simulink model "AircraftModel"  (R2025b)
settings: Solver=VariableStepAuto  StartTime=0.0  StopTime=200  RelTol=1e-3
InitFcn:
  | load("Aero.mat");
  | load("Prop.mat");
  | load("Motor.mat")
values from neighbouring files (symbols this model uses):
  A =     [Aero.mat]    (also in Aerodynamic.m = evalin("base", 'A'); QuaternionKinematics.m = [[0 -w(1) -w(2) -w(3)]; RotationalDynamics.m = evalin("base", "A"))
  Prop =     [Prop.mat]    (also in Propulsion.m = evalin("base", 'Prop'))
  WindAxes = [Va;a;b]    [Aerodynamic.m]
undefined symbols (not defined in the file or in its folder): Aerodynamic, Coordinates, Euler2Qbi, Euler2Rbi, EulerKinematics, Propulsion, Qbi2Euler, Qbi2Rbi, QuaternionKinematics, RotationalDynamics, WGS84
libraries: matrix_library x3, aerolibfltsims x2, simulink x1, aerolibatmos2 x1, sharedutil x1, aerosimlib x1
settings Model: Creator=User  LastModifiedBy=sutur
settings RTWCC: GPUComputeCapability=3.5

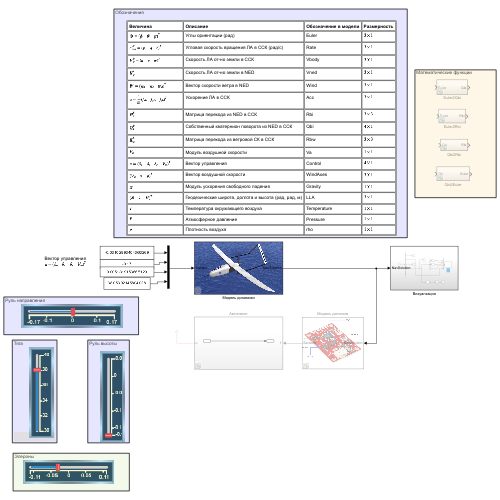
[thumbnail: Simulink's stored preview of the top-level diagram]
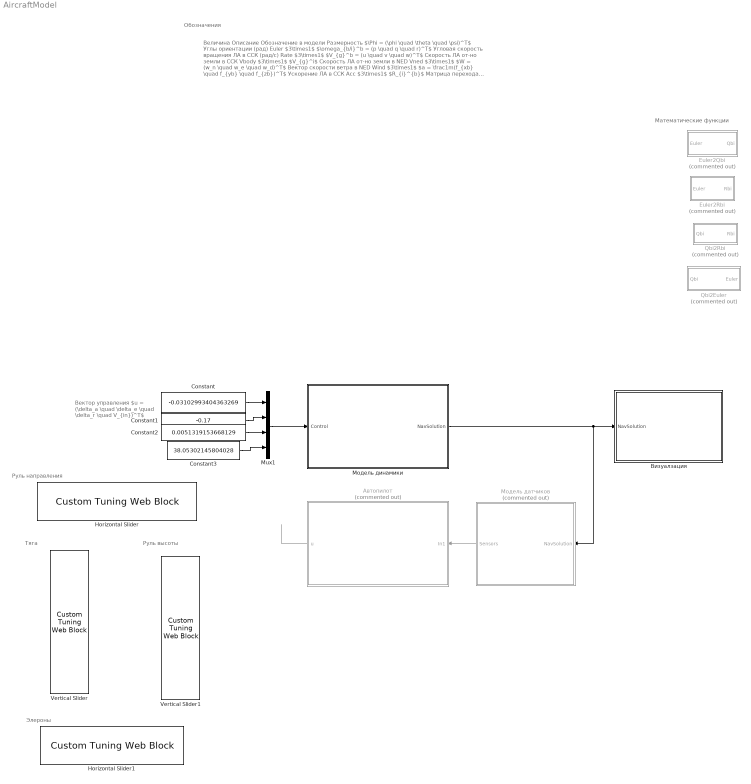
== system AircraftModel ==
  note: Руль направления
  note: Элероны
  note: Руль высоты
  note: Тяга
  note: Вектор управления
      | $u = (\delta_a \quad \delta_e \quad \delta_r \quad V_{in})^T$
  note: Математические функции
  note: Величина
      | Описание
      | Обозначение в модели
      | Размерность
      |
      | $\Phi = (\phi \quad \theta \quad \psi)^T$
      | Углы ориентации (рад)
      | Euler
      | $3\times1$
      |
      | $\omega_{b/i}^b = (p \quad q \quad r)^T$
      | Угловая скорость вращения ЛА в ССК (рад/с)
      | Rate
      | $3\times1$
      |
      | $V_{g}^b = (u \quad v \quad w)^T$
      | Скорость ЛА от-но земли в ССК
      | Vbody
      | $3\times1$
      |
      | $V_{g}^i$
      | Скорость ЛА от-но земли в NED
      | Vned
      | $3\times1$
      |
      | $W = (w_n \quad w_e \quad w_d)^T$
      | Вектор скорости ветра в NED
      | Wind
      | $3\times1$
      |
      | $a = \frac1m(f_{xb} \quad f_{yb} \quad f_{zb})^T$
      | Ускорение ЛА в ССК
      | Acc
      | $3\times1$
      |
      | $R_{i}^{b}$
      | Матрица перехода из NED в ССК
      | Rbi
      | $3\times3$
      |
      | $Q_{i}^{b}$
      | Собственный кватернион поворота из NED в ССК
      | Qbi
      | $4\times1$
      |
      | $R_w^b$
      | Матрица перехода из ветровой СК в ССК
      | Rbw
      | $3\times3$
      |
      | $V_a$
      | Модуль воздушной скорости
      | Va
      | $1\times1$
      |
      | $u = (\delta_a \quad \delta_e \quad \delta_r \quad V_{in})^T$
      | Вектор управления
      | Control
      | $4\times1$
      |
      | $(V_a \quad \alpha \quad \beta)^T$
      | Вектор воздушной скорости
      | WindAxes
      | $3\times1$
      |
      | $g$
      | Модуль ускорения свободного падения
      | Gravity
      | $1\times1$
      |
      | $(\phi \quad \lambda \quad H)^T$
      | Геодезические широта, долгота и высота (рад, рад, м)
      | LLA
      | $3\times1$
      |
      | $T$
      | Температура окружающего воздуха
      | Temperature
      | $1\times1$
      |
      | $P$
      | Атмосферное давление
      | Pressure
      | $1\times1$
      |
      | $\rho$
      | Плотность воздуха
      | rho
      | $1\times1$
  note: Обозначения
  Constant : Constant  Value=-0.03102993404363269
  Constant1 : Constant  Value=-0.17
  Constant2 : Constant  Value=0.0051319153668129
  Constant3 : Constant  Value=38.05302145804028
  Euler2Qbi : Subsystem  Commented=on
  Euler2Rbi : Subsystem  Commented=on
  Horizontal Slider : CustomTuningWebBlock  LabelPosition=Hide  ShowInitialText=on  Configuration="{\"components\":[{\"name\":\"LinearScaleComponent\",\"settings\":{\"bounds\":{\"max\":0.17,\"min\":-0.17,\"tickInterval\":\"auto\"},\"internalTickHeightScaleFactor\":0.5,\"labelColor\":[255,255,200],\"labelFont\":{\"font\":\"Arial\",\"fontSize\":12},\"labelOffset\":0.05,\"labelTransparency\":1,\"needleImage\":{\"size\":[596,842],\"src\":\"data:image\\/svg+xml;base64,PD94bWwgdmVyc2lvbj0iMS4wIiBlbmNvZGluZz0idXRmLTgiPz4NCjwhLS0gR2VuZXJhdG9yOiBBZG9iZSBJbGx1c3RyYXRvciAyNS4wLjAsIFNWRyBFeHBvcnQgUGx1Zy1JbiAuIFNWRyBWZXJzaW9uOiA2LjAwIEJ1aWxkIDApICAtLT4NCjxzdmcgdmVyc2lvbj0iMS4xIg0KCSBpZD0ic3ZnOCIgeG1sbnM6Y2M9Imh0dHA6Ly9jcmVhdGl2ZWNvbW1vbnMub3JnL25zIyIgeG1sbnM6ZGM9Imh0dHA6Ly9wdXJsLm9yZy9kYy9lbGVtZW50cy8xLjEvIiB4bWxuczppbmtzY2FwZT0iaHR0cDovL3d3dy5pbmtzY2FwZS5vcmcvbmFtZXNw ...(+2420 chars)\",\"srcOrientation\":\"Right\"},\"needleOffset\":[-0.8044596912521441,-0.0642123287671233],\"needleSize\":{\"height\":0.4337797619047619,\"width\":0.07668067226890757},\"position\":[0.2829861111111111,0.04398634453781513,0.9196428571428571,0.6088789682539683],\"referencePoint\":\"auto\",\"scaleColors\":[],\"scaleColorsSize\":0.2,\"scaleDirection\":\"LR\",\"showLabels\":1,\"showMinorTicks\":0,\"showSpanLine\":1,\"showTicks\":1,\"tickColor\":[252,252,197],\"tickTransparency\":1,\"valueBarColor\":[0,114,189],\"valueBarOffset\":-0.27,\"valueBarSize\":0.1,\"valueBarTransparency\":1}},{\"name\":\"BackgroundImageComponent\",\"settings\":{\"image\":{\"size\":[380,101],\"src\":\"data:image\\/svg+xml;base64,PHN2ZyB4bWxucz0iaHR0cDovL3d3dy53My5vcmcvMjAwMC9zdmciIHhtbG5zOnhsaW5rPSJodHRwOi8vd3d3LnczLm9yZy8xOTk5L3hsaW5rIiB2aWV3Qm94PSIwIDAgMzgwIDEwMSI+PGRlZnM+PHN0eWxlPi5jbHMtMXtmaWxsOiMwMDJiNDI7fS5jbHMtMntmaWxsOiM0MjcwODI7fS5jbHMtM3tmaWxsOnVybCgjcmFkaWFsLWdyYWRpZW50KTt9LmNscy00e2ZpbGw6I2M4YzhjODtzdHJva2U6IzAwMDt9PC9zdHlsZT48cmFkaWFsR3JhZGllbnQgaWQ9InJhZGlhbC1ncmFkaWVudCIgY3g9IjE5MCIgY3k9IjUwLjUiIHI9IjI2OS4yMSIgZ3JhZGllbnRVbml0cz0idXNlclNwYWNlT25Vc2UiPjxzdG9wIG9mZnNldD0iMC4wMSIgc3RvcC1jb2xvcj0iIzNlNGY1OCIvPjxzdG9wIG9mZnNldD0iMC4wNiIgc3RvcC1jb2xvcj0iIzQ0NTc2MSIvPjxzdG9wIG9mZnNldD0iMC4xNSIgc3RvcC1jb2xvcj0iIzU1NmE3NiIvPjxzdG9wIG9mZnNldD0iMC4yNSIgc3RvcC1jb2xvcj0iIzZkODg5NSIvPjxzdG9wIG9mZnNldD0iMC4zOCIgc3RvcC1jb2xvcj0iIzhmYjJjMyIvPjxzdG9wIG9mZnNldD0iMC41MiIgc3RvcC1jb2xvcj0iI2I2ZTRmYSIvPjxzdG9wIG9mZnNldD0iMSIgc3RvcC1jb2xvcj0iIzE1NDY1NyIvPjwvcmFkaWFsR3JhZGllbnQ+PC9kZWZzPjxnIGlkPSJmcmFtZSI+PGcgaWQ9IkxheWVyXzIiIGRhdGEtbmFtZT0iTGF5ZXIgMiI+PGcgaWQ9IkxheWVyXzEtMiIgZGF0YS1uYW1lPSJMYXllciAxLTIiPjxyZWN0IGlkPSJyZWN0MTAzNiIgY2xhc3M9ImNscy0xIiB4PSIxMSIgeT0iMTEiIHdpZHRoPSIzNTgiIGhlaWdodD0iNzkiLz48cGF0aCBpZD0icGF0aDEwMzgiIGNsYXNzPSJjbHMtMiIgZD0iTTgsOFY5M0gzNzJWOFpNMzY5LDkwSDExVjExSDM2OVoiLz48cGF0aCBpZD0icGF0aDEwNDAiIGNsYXNzPSJjbHMtMyIgZD0iTTAsMFYxMDFIMzgwVjBaTTM3Miw5M0g4VjhIMzcyWiIvPjwvZz48L2c+PC9nPjxnIGlkPSJ0cmFjayI+PHBhdGggaWQ9InJlY3QxNjExIiBjbGFzcz0iY2xzLTQiIGQ9Ik0zMy4zNywyNi41OUgzNDYuNjNjNCwwLDcuMjUsMi42LDcuMjUsNS44MWgwYzAsMy4yMS0zLjI1LDUuODItNy4yNSw1LjgySDMzLjM3Yy00LDAtNy4yNS0yLjYxLTcuMjUtNS44MmgwQzI2LjEyLDI5LjE5LDI5LjM3LDI2LjU5LDMzLjM3LDI2LjU5WiIvPjwvZz48L3N2Zz4=\",\"srcOrientation\":\"horizontal\"},\"position\":[0,0,1,1],\"scaleMode\":\"0\"}},{\"name\":\"ForegroundImageComponent\",\"settings\":{\"image\":{\"size\":[0,0],\"src\":\"default\",\"srcOrientation\":[]},\"isForeground\":1,\"position\":[0,0,1,1],\"scaleMode\":\"0\"}}],\"derived\":{\"blockParameters\":{\"ForegroundColor\":[0.9882352941176471,0.9882352941176471,0.7725490196078432],\"Limits\":{\"Max\":0.17,\"Min\":-0.17,\"Ticks\":\"auto\"},\"ScaleColors\":[],\"ScaleDirection\":\"Clockwise\",\"ScaleMax\":0.17,\"ScaleMin\":-0.17,\"TickInterval\":\"auto\",\"fixedAspectRatio\":\"on\"}},\"settings\":{\"BindingType\":\"param\",\"aspectRatio\":3.7777777777777777,\"backgroundColor\":[0,0,0,\"1\"],\"backgroundOffset\":0,\"backgroundOpacity\":1,\"fixedAspectRatio\":\"on\",\"foregroundColor\":[252,252,196],\"orientation\":\"horizontal\",\"showBackgroundColor\":false,\"value\":0,\"version\":\"R2023a\"},\"type\":\"LinearGauge\"}"
  Horizontal Slider1 : CustomTuningWebBlock  LabelPosition=Hide  ShowInitialText=on  Configuration="{\"components\":[{\"name\":\"LinearScaleComponent\",\"settings\":{\"bounds\":{\"max\":0.11,\"min\":-0.11,\"tickInterval\":\"auto\"},\"internalTickHeightScaleFactor\":0.5,\"labelColor\":[255,255,200],\"labelFont\":{\"font\":\"Arial\",\"fontSize\":12},\"labelOffset\":0.05,\"labelTransparency\":1,\"needleImage\":{\"size\":[596,842],\"src\":\"data:image\\/svg+xml;base64,PD94bWwgdmVyc2lvbj0iMS4wIiBlbmNvZGluZz0idXRmLTgiPz4NCjwhLS0gR2VuZXJhdG9yOiBBZG9iZSBJbGx1c3RyYXRvciAyNS4wLjAsIFNWRyBFeHBvcnQgUGx1Zy1JbiAuIFNWRyBWZXJzaW9uOiA2LjAwIEJ1aWxkIDApICAtLT4NCjxzdmcgdmVyc2lvbj0iMS4xIg0KCSBpZD0ic3ZnOCIgeG1sbnM6Y2M9Imh0dHA6Ly9jcmVhdGl2ZWNvbW1vbnMub3JnL25zIyIgeG1sbnM6ZGM9Imh0dHA6Ly9wdXJsLm9yZy9kYy9lbGVtZW50cy8xLjEvIiB4bWxuczppbmtzY2FwZT0iaHR0cDovL3d3dy5pbmtzY2FwZS5vcmcvbmFtZXNw ...(+2420 chars)\",\"srcOrientation\":\"Right\"},\"needleOffset\":[-0.8044596912521441,-0.0642123287671233],\"needleSize\":{\"height\":0.4337797619047619,\"width\":0.07668067226890757},\"position\":[0.2829861111111111,0.04398634453781513,0.9196428571428571,0.6088789682539683],\"referencePoint\":\"auto\",\"scaleColors\":[],\"scaleColorsSize\":0.2,\"scaleDirection\":\"LR\",\"showLabels\":1,\"showMinorTicks\":0,\"showSpanLine\":1,\"showTicks\":1,\"tickColor\":[252,252,197],\"tickTransparency\":1,\"valueBarColor\":[0,114,189],\"valueBarOffset\":-0.27,\"valueBarSize\":0.1,\"valueBarTransparency\":1}},{\"name\":\"BackgroundImageComponent\",\"settings\":{\"image\":{\"size\":[380,101],\"src\":\"data:image\\/svg+xml;base64,PHN2ZyB4bWxucz0iaHR0cDovL3d3dy53My5vcmcvMjAwMC9zdmciIHhtbG5zOnhsaW5rPSJodHRwOi8vd3d3LnczLm9yZy8xOTk5L3hsaW5rIiB2aWV3Qm94PSIwIDAgMzgwIDEwMSI+PGRlZnM+PHN0eWxlPi5jbHMtMXtmaWxsOiMwMDJiNDI7fS5jbHMtMntmaWxsOiM0MjcwODI7fS5jbHMtM3tmaWxsOnVybCgjcmFkaWFsLWdyYWRpZW50KTt9LmNscy00e2ZpbGw6I2M4YzhjODtzdHJva2U6IzAwMDt9PC9zdHlsZT48cmFkaWFsR3JhZGllbnQgaWQ9InJhZGlhbC1ncmFkaWVudCIgY3g9IjE5MCIgY3k9IjUwLjUiIHI9IjI2OS4yMSIgZ3JhZGllbnRVbml0cz0idXNlclNwYWNlT25Vc2UiPjxzdG9wIG9mZnNldD0iMC4wMSIgc3RvcC1jb2xvcj0iIzNlNGY1OCIvPjxzdG9wIG9mZnNldD0iMC4wNiIgc3RvcC1jb2xvcj0iIzQ0NTc2MSIvPjxzdG9wIG9mZnNldD0iMC4xNSIgc3RvcC1jb2xvcj0iIzU1NmE3NiIvPjxzdG9wIG9mZnNldD0iMC4yNSIgc3RvcC1jb2xvcj0iIzZkODg5NSIvPjxzdG9wIG9mZnNldD0iMC4zOCIgc3RvcC1jb2xvcj0iIzhmYjJjMyIvPjxzdG9wIG9mZnNldD0iMC41MiIgc3RvcC1jb2xvcj0iI2I2ZTRmYSIvPjxzdG9wIG9mZnNldD0iMSIgc3RvcC1jb2xvcj0iIzE1NDY1NyIvPjwvcmFkaWFsR3JhZGllbnQ+PC9kZWZzPjxnIGlkPSJmcmFtZSI+PGcgaWQ9IkxheWVyXzIiIGRhdGEtbmFtZT0iTGF5ZXIgMiI+PGcgaWQ9IkxheWVyXzEtMiIgZGF0YS1uYW1lPSJMYXllciAxLTIiPjxyZWN0IGlkPSJyZWN0MTAzNiIgY2xhc3M9ImNscy0xIiB4PSIxMSIgeT0iMTEiIHdpZHRoPSIzNTgiIGhlaWdodD0iNzkiLz48cGF0aCBpZD0icGF0aDEwMzgiIGNsYXNzPSJjbHMtMiIgZD0iTTgsOFY5M0gzNzJWOFpNMzY5LDkwSDExVjExSDM2OVoiLz48cGF0aCBpZD0icGF0aDEwNDAiIGNsYXNzPSJjbHMtMyIgZD0iTTAsMFYxMDFIMzgwVjBaTTM3Miw5M0g4VjhIMzcyWiIvPjwvZz48L2c+PC9nPjxnIGlkPSJ0cmFjayI+PHBhdGggaWQ9InJlY3QxNjExIiBjbGFzcz0iY2xzLTQiIGQ9Ik0zMy4zNywyNi41OUgzNDYuNjNjNCwwLDcuMjUsMi42LDcuMjUsNS44MWgwYzAsMy4yMS0zLjI1LDUuODItNy4yNSw1LjgySDMzLjM3Yy00LDAtNy4yNS0yLjYxLTcuMjUtNS44MmgwQzI2LjEyLDI5LjE5LDI5LjM3LDI2LjU5LDMzLjM3LDI2LjU5WiIvPjwvZz48L3N2Zz4=\",\"srcOrientation\":\"horizontal\"},\"position\":[0,0,1,1],\"scaleMode\":\"0\"}},{\"name\":\"ForegroundImageComponent\",\"settings\":{\"image\":{\"size\":[0,0],\"src\":\"default\",\"srcOrientation\":[]},\"isForeground\":1,\"position\":[0,0,1,1],\"scaleMode\":\"0\"}}],\"derived\":{\"blockParameters\":{\"ForegroundColor\":[0.9882352941176471,0.9882352941176471,0.7725490196078432],\"Limits\":{\"Max\":0.11,\"Min\":-0.11,\"Ticks\":\"auto\"},\"ScaleColors\":[],\"ScaleDirection\":\"Clockwise\",\"ScaleMax\":0.11,\"ScaleMin\":-0.11,\"TickInterval\":\"auto\",\"fixedAspectRatio\":\"on\"}},\"settings\":{\"BindingType\":\"param\",\"aspectRatio\":3.7777777777777777,\"backgroundColor\":[0,0,0,\"1\"],\"backgroundOffset\":0,\"backgroundOpacity\":1,\"fixedAspectRatio\":\"on\",\"foregroundColor\":[252,252,196],\"orientation\":\"horizontal\",\"showBackgroundColor\":false,\"value\":0,\"version\":\"R2023a\"},\"type\":\"LinearGauge\"}"
  Mux1 : Mux
  Qbi2Euler : Subsystem  Commented=on
  Qbi2Rbi : Subsystem  Commented=on
  Vertical Slider : CustomTuningWebBlock  LabelPosition=Hide  ShowInitialText=on  Configuration="{\"components\":[{\"name\":\"LinearScaleComponent\",\"settings\":{\"bounds\":{\"max\":40,\"min\":30,\"tickInterval\":\"auto\"},\"internalTickHeightScaleFactor\":0.5,\"labelColor\":[255,255,200],\"labelFont\":{\"font\":\"Arial\",\"fontSize\":12},\"labelOffset\":0.05,\"labelTransparency\":1,\"needleImage\":{\"size\":[596,842],\"src\":\"data:image\\/svg+xml;base64,PD94bWwgdmVyc2lvbj0iMS4wIiBlbmNvZGluZz0idXRmLTgiPz4NCjwhLS0gR2VuZXJhdG9yOiBBZG9iZSBJbGx1c3RyYXRvciAyNS4wLjAsIFNWRyBFeHBvcnQgUGx1Zy1JbiAuIFNWRyBWZXJzaW9uOiA2LjAwIEJ1aWxkIDApICAtLT4NCjxzdmcgdmVyc2lvbj0iMS4xIg0KCSBpZD0ic3ZnOCIgeG1sbnM6Y2M9Imh0dHA6Ly9jcmVhdGl2ZWNvbW1vbnMub3JnL25zIyIgeG1sbnM6ZGM9Imh0dHA6Ly9wdXJsLm9yZy9kYy9lbGVtZW50cy8xLjEvIiB4bWxuczppbmtzY2FwZT0iaHR0cDovL3d3dy5pbmtzY2FwZS5vcmcvbmFtZXNw ...(+2420 chars)\",\"srcOrientation\":\"horizontal\"},\"needleOffset\":[0.0642123287671233,-0.8044596912521441],\"needleSize\":{\"height\":0.07668067226890757,\"width\":0.4337797619047619},\"position\":[0.03623949579831933,0.2829861111111111,0.6088789682539683,0.9196428571428571],\"referencePoint\":\"auto\",\"scaleColors\":[],\"scaleColorsSize\":0.2,\"scaleDirection\":\"BT\",\"showLabels\":1,\"showMinorTicks\":0,\"showSpanLine\":1,\"showTicks\":1,\"tickColor\":[252,252,197],\"tickTransparency\":1,\"valueBarColor\":[0,114,189],\"valueBarOffset\":-0.27,\"valueBarSize\":0.1,\"valueBarTransparency\":1}},{\"name\":\"BackgroundImageComponent\",\"settings\":{\"image\":{\"size\":[380,101],\"src\":\"data:image\\/svg+xml;base64,PHN2ZyB4bWxucz0iaHR0cDovL3d3dy53My5vcmcvMjAwMC9zdmciIHhtbG5zOnhsaW5rPSJodHRwOi8vd3d3LnczLm9yZy8xOTk5L3hsaW5rIiB2aWV3Qm94PSIwIDAgMzgwIDEwMSI+PGRlZnM+PHN0eWxlPi5jbHMtMXtmaWxsOiMwMDJiNDI7fS5jbHMtMntmaWxsOiM0MjcwODI7fS5jbHMtM3tmaWxsOnVybCgjcmFkaWFsLWdyYWRpZW50KTt9LmNscy00e2ZpbGw6I2M4YzhjODtzdHJva2U6IzAwMDt9PC9zdHlsZT48cmFkaWFsR3JhZGllbnQgaWQ9InJhZGlhbC1ncmFkaWVudCIgY3g9IjE5MCIgY3k9IjUwLjUiIHI9IjI2OS4yMSIgZ3JhZGllbnRVbml0cz0idXNlclNwYWNlT25Vc2UiPjxzdG9wIG9mZnNldD0iMC4wMSIgc3RvcC1jb2xvcj0iIzNlNGY1OCIvPjxzdG9wIG9mZnNldD0iMC4wNiIgc3RvcC1jb2xvcj0iIzQ0NTc2MSIvPjxzdG9wIG9mZnNldD0iMC4xNSIgc3RvcC1jb2xvcj0iIzU1NmE3NiIvPjxzdG9wIG9mZnNldD0iMC4yNSIgc3RvcC1jb2xvcj0iIzZkODg5NSIvPjxzdG9wIG9mZnNldD0iMC4zOCIgc3RvcC1jb2xvcj0iIzhmYjJjMyIvPjxzdG9wIG9mZnNldD0iMC41MiIgc3RvcC1jb2xvcj0iI2I2ZTRmYSIvPjxzdG9wIG9mZnNldD0iMSIgc3RvcC1jb2xvcj0iIzE1NDY1NyIvPjwvcmFkaWFsR3JhZGllbnQ+PC9kZWZzPjxnIGlkPSJmcmFtZSI+PGcgaWQ9IkxheWVyXzIiIGRhdGEtbmFtZT0iTGF5ZXIgMiI+PGcgaWQ9IkxheWVyXzEtMiIgZGF0YS1uYW1lPSJMYXllciAxLTIiPjxyZWN0IGlkPSJyZWN0MTAzNiIgY2xhc3M9ImNscy0xIiB4PSIxMSIgeT0iMTEiIHdpZHRoPSIzNTgiIGhlaWdodD0iNzkiLz48cGF0aCBpZD0icGF0aDEwMzgiIGNsYXNzPSJjbHMtMiIgZD0iTTgsOFY5M0gzNzJWOFpNMzY5LDkwSDExVjExSDM2OVoiLz48cGF0aCBpZD0icGF0aDEwNDAiIGNsYXNzPSJjbHMtMyIgZD0iTTAsMFYxMDFIMzgwVjBaTTM3Miw5M0g4VjhIMzcyWiIvPjwvZz48L2c+PC9nPjxnIGlkPSJ0cmFjayI+PHBhdGggaWQ9InJlY3QxNjExIiBjbGFzcz0iY2xzLTQiIGQ9Ik0zMy4zNywyNi41OUgzNDYuNjNjNCwwLDcuMjUsMi42LDcuMjUsNS44MWgwYzAsMy4yMS0zLjI1LDUuODItNy4yNSw1LjgySDMzLjM3Yy00LDAtNy4yNS0yLjYxLTcuMjUtNS44MmgwQzI2LjEyLDI5LjE5LDI5LjM3LDI2LjU5LDMzLjM3LDI2LjU5WiIvPjwvZz48L3N2Zz4=\",\"srcOrientation\":\"horizontal\"},\"position\":[0,0,1,1],\"scaleMode\":\"0\"}},{\"name\":\"ForegroundImageComponent\",\"settings\":{\"image\":{\"size\":[0,0],\"src\":\"default\",\"srcOrientation\":[]},\"isForeground\":1,\"position\":[0,0,1,1],\"scaleMode\":\"0\"}}],\"derived\":{\"blockParameters\":{\"ForegroundColor\":[0.9882352941176471,0.9882352941176471,0.7725490196078432],\"Limits\":{\"Max\":40,\"Min\":30,\"Ticks\":\"auto\"},\"ScaleColors\":[],\"ScaleDirection\":\"Clockwise\",\"ScaleMax\":40,\"ScaleMin\":30,\"TickInterval\":\"auto\",\"fixedAspectRatio\":\"on\"}},\"settings\":{\"BindingType\":\"param\",\"aspectRatio\":3.7777777777777777,\"backgroundColor\":[0,0,0,\"1\"],\"backgroundOffset\":0,\"backgroundOpacity\":1,\"fixedAspectRatio\":\"on\",\"foregroundColor\":[252,252,196],\"orientation\":\"vertical\",\"showBackgroundColor\":false,\"value\":0,\"version\":\"R2023a\"},\"type\":\"LinearGauge\"}"
  Vertical Slider1 : CustomTuningWebBlock  LabelPosition=Hide  ShowInitialText=on  Configuration="{\"components\":[{\"name\":\"LinearScaleComponent\",\"settings\":{\"bounds\":{\"max\":0.05,\"min\":-0.17,\"tickInterval\":\"auto\"},\"internalTickHeightScaleFactor\":0.5,\"labelColor\":[255,255,200],\"labelFont\":{\"font\":\"Arial\",\"fontSize\":12},\"labelOffset\":0.05,\"labelTransparency\":1,\"needleImage\":{\"size\":[596,842],\"src\":\"data:image\\/svg+xml;base64,PD94bWwgdmVyc2lvbj0iMS4wIiBlbmNvZGluZz0idXRmLTgiPz4NCjwhLS0gR2VuZXJhdG9yOiBBZG9iZSBJbGx1c3RyYXRvciAyNS4wLjAsIFNWRyBFeHBvcnQgUGx1Zy1JbiAuIFNWRyBWZXJzaW9uOiA2LjAwIEJ1aWxkIDApICAtLT4NCjxzdmcgdmVyc2lvbj0iMS4xIg0KCSBpZD0ic3ZnOCIgeG1sbnM6Y2M9Imh0dHA6Ly9jcmVhdGl2ZWNvbW1vbnMub3JnL25zIyIgeG1sbnM6ZGM9Imh0dHA6Ly9wdXJsLm9yZy9kYy9lbGVtZW50cy8xLjEvIiB4bWxuczppbmtzY2FwZT0iaHR0cDovL3d3dy5pbmtzY2FwZS5vcmcvbmFtZXNw ...(+2420 chars)\",\"srcOrientation\":\"horizontal\"},\"needleOffset\":[0.0642123287671233,-0.8044596912521441],\"needleSize\":{\"height\":0.07668067226890757,\"width\":0.4337797619047619},\"position\":[0.03623949579831933,0.2829861111111111,0.6088789682539683,0.9196428571428571],\"referencePoint\":\"auto\",\"scaleColors\":[],\"scaleColorsSize\":0.2,\"scaleDirection\":\"BT\",\"showLabels\":1,\"showMinorTicks\":0,\"showSpanLine\":1,\"showTicks\":1,\"tickColor\":[252,252,197],\"tickTransparency\":1,\"valueBarColor\":[0,114,189],\"valueBarOffset\":-0.27,\"valueBarSize\":0.1,\"valueBarTransparency\":1}},{\"name\":\"BackgroundImageComponent\",\"settings\":{\"image\":{\"size\":[380,101],\"src\":\"data:image\\/svg+xml;base64,PHN2ZyB4bWxucz0iaHR0cDovL3d3dy53My5vcmcvMjAwMC9zdmciIHhtbG5zOnhsaW5rPSJodHRwOi8vd3d3LnczLm9yZy8xOTk5L3hsaW5rIiB2aWV3Qm94PSIwIDAgMzgwIDEwMSI+PGRlZnM+PHN0eWxlPi5jbHMtMXtmaWxsOiMwMDJiNDI7fS5jbHMtMntmaWxsOiM0MjcwODI7fS5jbHMtM3tmaWxsOnVybCgjcmFkaWFsLWdyYWRpZW50KTt9LmNscy00e2ZpbGw6I2M4YzhjODtzdHJva2U6IzAwMDt9PC9zdHlsZT48cmFkaWFsR3JhZGllbnQgaWQ9InJhZGlhbC1ncmFkaWVudCIgY3g9IjE5MCIgY3k9IjUwLjUiIHI9IjI2OS4yMSIgZ3JhZGllbnRVbml0cz0idXNlclNwYWNlT25Vc2UiPjxzdG9wIG9mZnNldD0iMC4wMSIgc3RvcC1jb2xvcj0iIzNlNGY1OCIvPjxzdG9wIG9mZnNldD0iMC4wNiIgc3RvcC1jb2xvcj0iIzQ0NTc2MSIvPjxzdG9wIG9mZnNldD0iMC4xNSIgc3RvcC1jb2xvcj0iIzU1NmE3NiIvPjxzdG9wIG9mZnNldD0iMC4yNSIgc3RvcC1jb2xvcj0iIzZkODg5NSIvPjxzdG9wIG9mZnNldD0iMC4zOCIgc3RvcC1jb2xvcj0iIzhmYjJjMyIvPjxzdG9wIG9mZnNldD0iMC41MiIgc3RvcC1jb2xvcj0iI2I2ZTRmYSIvPjxzdG9wIG9mZnNldD0iMSIgc3RvcC1jb2xvcj0iIzE1NDY1NyIvPjwvcmFkaWFsR3JhZGllbnQ+PC9kZWZzPjxnIGlkPSJmcmFtZSI+PGcgaWQ9IkxheWVyXzIiIGRhdGEtbmFtZT0iTGF5ZXIgMiI+PGcgaWQ9IkxheWVyXzEtMiIgZGF0YS1uYW1lPSJMYXllciAxLTIiPjxyZWN0IGlkPSJyZWN0MTAzNiIgY2xhc3M9ImNscy0xIiB4PSIxMSIgeT0iMTEiIHdpZHRoPSIzNTgiIGhlaWdodD0iNzkiLz48cGF0aCBpZD0icGF0aDEwMzgiIGNsYXNzPSJjbHMtMiIgZD0iTTgsOFY5M0gzNzJWOFpNMzY5LDkwSDExVjExSDM2OVoiLz48cGF0aCBpZD0icGF0aDEwNDAiIGNsYXNzPSJjbHMtMyIgZD0iTTAsMFYxMDFIMzgwVjBaTTM3Miw5M0g4VjhIMzcyWiIvPjwvZz48L2c+PC9nPjxnIGlkPSJ0cmFjayI+PHBhdGggaWQ9InJlY3QxNjExIiBjbGFzcz0iY2xzLTQiIGQ9Ik0zMy4zNywyNi41OUgzNDYuNjNjNCwwLDcuMjUsMi42LDcuMjUsNS44MWgwYzAsMy4yMS0zLjI1LDUuODItNy4yNSw1LjgySDMzLjM3Yy00LDAtNy4yNS0yLjYxLTcuMjUtNS44MmgwQzI2LjEyLDI5LjE5LDI5LjM3LDI2LjU5LDMzLjM3LDI2LjU5WiIvPjwvZz48L3N2Zz4=\",\"srcOrientation\":\"horizontal\"},\"position\":[0,0,1,1],\"scaleMode\":\"0\"}},{\"name\":\"ForegroundImageComponent\",\"settings\":{\"image\":{\"size\":[0,0],\"src\":\"default\",\"srcOrientation\":[]},\"isForeground\":1,\"position\":[0,0,1,1],\"scaleMode\":\"0\"}}],\"derived\":{\"blockParameters\":{\"ForegroundColor\":[0.9882352941176471,0.9882352941176471,0.7725490196078432],\"Limits\":{\"Max\":0.05,\"Min\":-0.17,\"Ticks\":\"auto\"},\"ScaleColors\":[],\"ScaleDirection\":\"Clockwise\",\"ScaleMax\":0.05,\"ScaleMin\":-0.17,\"TickInterval\":\"auto\",\"fixedAspectRatio\":\"on\"}},\"settings\":{\"BindingType\":\"param\",\"aspectRatio\":3.7777777777777777,\"backgroundColor\":[0,0,0,\"1\"],\"backgroundOffset\":0,\"backgroundOpacity\":1,\"fixedAspectRatio\":\"on\",\"foregroundColor\":[252,252,196],\"orientation\":\"vertical\",\"showBackgroundColor\":false,\"value\":0,\"version\":\"R2023a\"},\"type\":\"LinearGauge\"}"
  Автопилот : Subsystem  Commented=on
  Визуалзация : Subsystem
  Модель датчиков : Subsystem  Commented=on
      mask Display: image('IMU.jpg');
  Модель динамики : Subsystem  mask{InitVbody=[25;0;0], InitLLA=[deg2rad(53.675672);deg2rad(109.029085);1450], InitEuler=[0;1;0]*pi/180, InitRate=[0;0;0]*pi/180}
      mask prompts: InitVbody "Начальная скорость в ССК"; InitLLA "Начальное положение"; InitEuler "Начальная ориентация"; InitRate "Начальные угловый скорости"
      mask Display: image('Aerosonde.jpg');
  wires:
  Модель динамики/1(NavSolution) -> Модель датчиков/1(NavSolution), Визуалзация/1(NavSolution)
  Модель датчиков/1(Sensors) -> Автопилот/1(In1)
  Автопилот/1(u) -> ?
  Mux1/1 -> Модель динамики/1(Control)
  Constant/1 -> Mux1/1
  Constant1/1 -> Mux1/2
  Constant3/1 -> Mux1/4
  Constant2/1 -> Mux1/3

== system AircraftModel/Euler2Qbi ==
  Euler : Inport
  Interpreted MATLAB Function : MATLABFcn  MATLABFcn=Euler2Qbi(u)
  Qbi : Outport
  wires:
  Euler/1 -> Interpreted MATLAB Function/1
  Interpreted MATLAB Function/1 -> Qbi/1

== system AircraftModel/Euler2Rbi ==
  Euler : Inport
  Interpreted MATLAB Function : MATLABFcn  MATLABFcn=Euler2Rbi(u)
  Rbi : Outport
  wires:
  Euler/1 -> Interpreted MATLAB Function/1
  Interpreted MATLAB Function/1 -> Rbi/1

== system AircraftModel/Qbi2Euler ==
  Qbi : Inport
  Interpreted MATLAB Function : MATLABFcn  MATLABFcn=Qbi2Euler(u)
  Euler : Outport
  wires:
  Qbi/1 -> Interpreted MATLAB Function/1
  Interpreted MATLAB Function/1 -> Euler/1

== system AircraftModel/Qbi2Rbi ==
  Qbi : Inport
  Interpreted MATLAB Function : MATLABFcn  MATLABFcn=Qbi2Rbi(u)  Output1D=off
  Rbi : Outport
  wires:
  Qbi/1 -> Interpreted MATLAB Function/1
  Interpreted MATLAB Function/1 -> Rbi/1

== system AircraftModel/Автопилот ==
  In1 : Inport
  u : Outport
  wires:
  In1/1 -> u/1

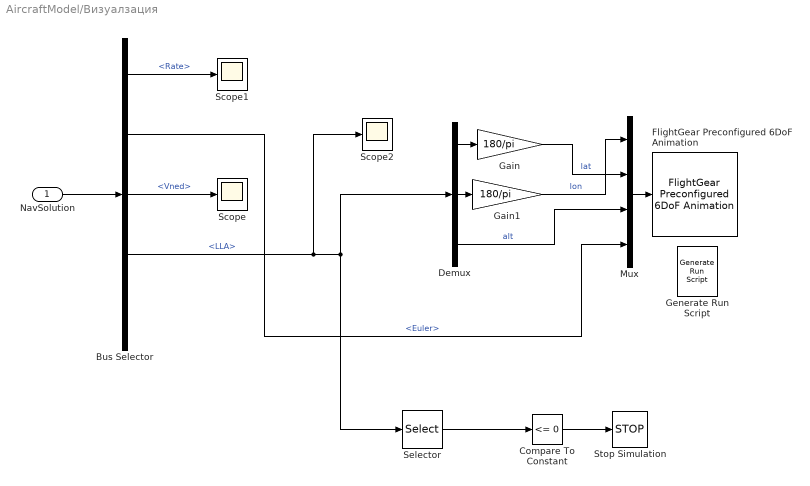
== system AircraftModel/Визуалзация ==
  NavSolution : Inport
  Bus Selector : BusSelector  OutputSignals=Rate,Euler,Vned,LLA,Position
  Compare To Constant : simulink/Logic and Bit Operations/Compare To Constant  relop=<=  const=0  OutDataTypeStr=boolean
  Demux : Demux  Outputs=3
  FlightGear Preconfigured 6DoF Animation : aerolibfltsims/FlightGear Preconfigured 6DoF Animation  xFlightGearVersion=v2019.1  DestinationIpAddress=127.0.0.1  DestinationPort=5502  SampleTime=1/30  packetVersion=24
  Gain : Gain  Gain=180/pi
  Gain1 : Gain  Gain=180/pi
  Generate Run Script : aerolibfltsims/Generate Run Script  Architecture=Win64  dataFlow=Send  GeometryModelName=c172p  AirportId=KSFO  RunwayId=10L  InitialAltitude=7224  InitialHeading=113  OffsetDistance=4.72  OffsetAzimuth=0  InstallScenery=off  DisableShaders=on  OriginAddress=127.0.0.1  DestinationPort=5502  OriginPort=5505  LocalAddress=127.0.0.1  OutputFileName=runfg.bat  FlightGearBaseDirectory=D:\Program Files\FlightGear 2024.1
  Mux : Mux
  Scope : Scope
      settings: ActiveDisplayYMinimum=-59.307455333700915  ActiveDisplayYMaximum=58.146276813191271  DataLoggingVariableName=ScopeData4
  Scope1 : Scope
      settings: DataLoggingVariableName=ScopeData5
  Scope2 : Scope
      settings: ActiveDisplayYMinimum=1465.7359510692422  ActiveDisplayYMaximum=1646.6843877725191  DataLoggingVariableName=ScopeData6
  Selector : Selector  InputPortWidth=3  IndexOptions=Index vector (dialog)  Indices=[3]  OutputSizes=1
  Stop Simulation : Stop
  wires:
  NavSolution/1 -> Bus Selector/1
  Demux/2 -> Gain1/1
  Demux/1 -> Gain/1
  Demux/3 -> Mux/3  "alt"
  Gain/1 -> Mux/2  "lat"
  Gain1/1 -> Mux/1  "lon"
  Mux/1 -> FlightGear Preconfigured 6DoF Animation/1
  Bus Selector/1 -> Scope1/1  "<Rate>"
  Bus Selector/2 -> Mux/4  "<Euler>"
  Bus Selector/3 -> Scope/1  "<Vned>"
  Bus Selector/4 -> Scope2/1, Selector/1, Demux/1  "<LLA>"
  Selector/1 -> Compare To Constant/1
  Compare To Constant/1 -> Stop Simulation/1

== system AircraftModel/Модель датчиков ==
  NavSolution : Inport
  Sensors : Outport
  wires:
  NavSolution/1 -> Sensors/1

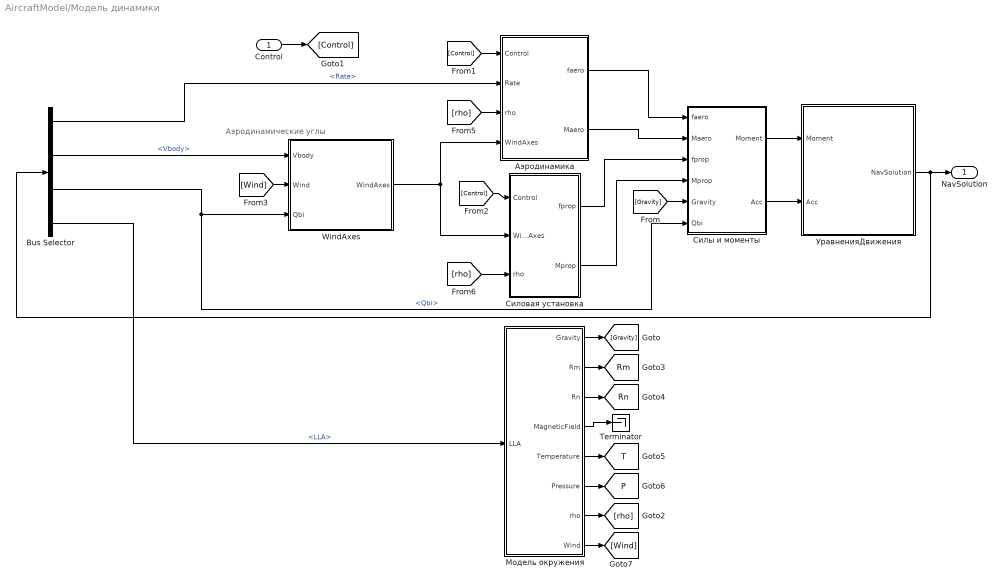
== system AircraftModel/Модель динамики ==
  note: Аэродинамические углы
  Control : Inport
  Bus Selector : BusSelector  OutputSignals=Rate,Vbody,Qbi,LLA
  Terminator : Terminator
  WindAxes : Subsystem
  Аэродинамика : Subsystem
  Модель окружения : Subsystem
  Силовая установка : Subsystem
  Силы и моменты : Subsystem
  УравненияДвижения : Subsystem
  NavSolution : Outport
  tag scope: P=global, Rm=global, Rn=global, T=global
  wires:
  УравненияДвижения/1(NavSolution) -> Bus Selector/1, NavSolution/1
  Аэродинамика/1(faero) -> Силы и моменты/1(faero)
  Аэродинамика/2(Maero) -> Силы и моменты/2(Maero)
  Силовая установка/1(fprop) -> Силы и моменты/3(fprop)
  Силовая установка/2(Mprop) -> Силы и моменты/4(Mprop)
  [Gravity] -> Силы и моменты/5(Gravity)
  Модель окружения/1(Gravity) -> [Gravity]
  Силы и моменты/2(Acc) -> УравненияДвижения/2(" Acc")
  Силы и моменты/1(Moment) -> УравненияДвижения/1(" Moment")
  Control/1 -> [Control]
  [Control] -> Силовая установка/1(Control)
  [Control] -> Аэродинамика/1(Control)
  [rho] -> Аэродинамика/3(rho)
  Модель окружения/7(rho) -> [rho]
  [rho] -> Силовая установка/3(rho)
  Модель окружения/2(Rm) -> [Rm]
  Модель окружения/3(Rn) -> [Rn]
  Модель окружения/5(Temperature) -> [T]
  Модель окружения/6(Pressure) -> [P]
  Модель окружения/8(Wind) -> [Wind]
  Модель окружения/4(MagneticField) -> Terminator/1
  Bus Selector/1 -> Аэродинамика/2(Rate)  "<Rate>"
  Bus Selector/3 -> WindAxes/3(Qbi), Силы и моменты/6(Qbi)  "<Qbi>"
  Bus Selector/2 -> WindAxes/1(Vbody)  "<Vbody>"
  WindAxes/1(WindAxes) -> Силовая установка/2(WindAxes), Аэродинамика/4(WindAxes)
  [Wind] -> WindAxes/2(Wind)
  Bus Selector/4 -> Модель окружения/1(LLA)  "<LLA>"

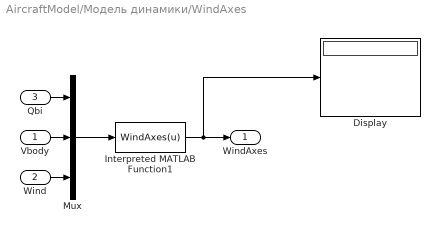
== system AircraftModel/Модель динамики/WindAxes ==
  Vbody : Inport
  Wind : Inport  Port=2
  Qbi : Inport  Port=3
  Display : Display
  Interpreted MATLAB Function1 : MATLABFcn  MATLABFcn=WindAxes(u)
  Mux : Mux  Inputs=3
  WindAxes : Outport
  wires:
  Qbi/1 -> Mux/1
  Mux/1 -> Interpreted MATLAB Function1/1
  Interpreted MATLAB Function1/1 -> Display/1, WindAxes/1
  Vbody/1 -> Mux/2
  Wind/1 -> Mux/3

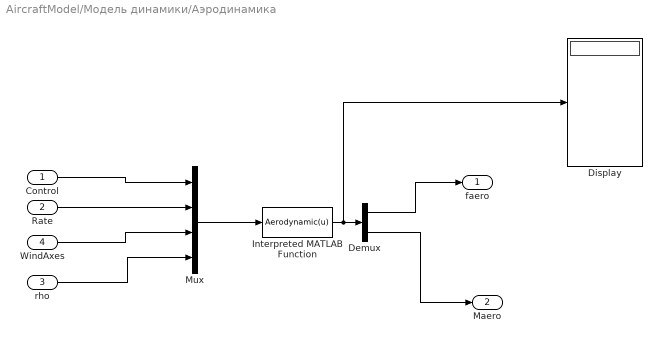
== system AircraftModel/Модель динамики/Аэродинамика ==
  Control : Inport
  Rate : Inport  Port=2
  rho : Inport  Port=3
  WindAxes : Inport  Port=4
  Demux : Demux  Outputs=2
  Display : Display
  Interpreted MATLAB Function : MATLABFcn  MATLABFcn=Aerodynamic(u)
  Mux : Mux
  faero : Outport
  Maero : Outport  Port=2
  wires:
  Control/1 -> Mux/1
  Demux/1 -> faero/1
  Demux/2 -> Maero/1
  Mux/1 -> Interpreted MATLAB Function/1
  Rate/1 -> Mux/2
  Interpreted MATLAB Function/1 -> Display/1, Demux/1
  rho/1 -> Mux/4
  WindAxes/1 -> Mux/3

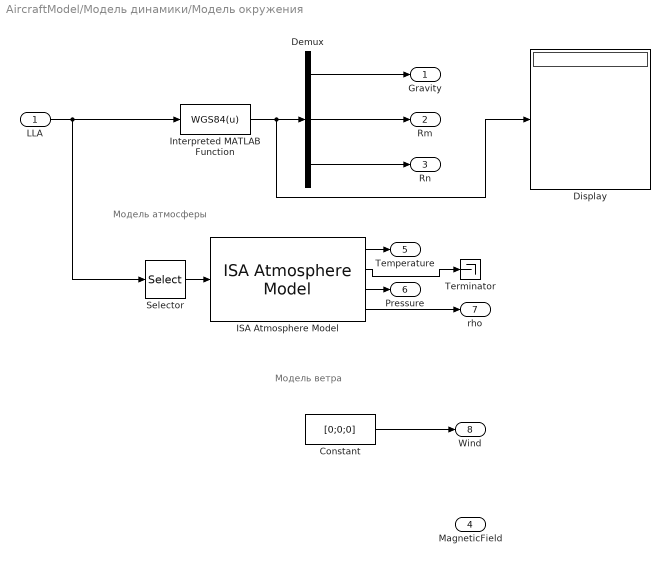
== system AircraftModel/Модель динамики/Модель окружения ==
  note: Модель ветра
  note: Модель атмосферы
  LLA : Inport
  Constant : Constant  Value=[0;0;0]
  Demux : Demux  Outputs=3
  Display : Display
  ISA Atmosphere Model : aerolibatmos2/ISA Atmosphere Model  useExtended=off  action=None  custom=off  viscosityOut=off  g=9.80665  gamma=1.4  R=287.0531  L=0.0065  h_trop=11000  h_strat=20000  rho0=1.225  P0=101325  T0=288.15  h0=0  S=110.4  Tref=273.15  muref=1.716e-5
  Interpreted MATLAB Function : MATLABFcn  MATLABFcn=WGS84(u)
  Selector : Selector  InputPortWidth=3  IndexOptions=Index vector (dialog)  Indices=[3]  OutputSizes=1
  Terminator : Terminator
  Gravity : Outport
  Rm : Outport  Port=2
  Rn : Outport  Port=3
  MagneticField : Outport  Port=4
  Temperature : Outport  Port=5
  Pressure : Outport  Port=6
  rho : Outport  Port=7
  Wind : Outport  Port=8
  wires:
  LLA/1 -> Selector/1, Interpreted MATLAB Function/1
  Selector/1 -> ISA Atmosphere Model/1
  ISA Atmosphere Model/1 -> Temperature/1
  ISA Atmosphere Model/3 -> Pressure/1
  ISA Atmosphere Model/4 -> rho/1
  Interpreted MATLAB Function/1 -> Display/1, Demux/1
  Demux/1 -> Gravity/1
  Demux/2 -> Rm/1
  Demux/3 -> Rn/1
  ISA Atmosphere Model/2 -> Terminator/1
  Constant/1 -> Wind/1

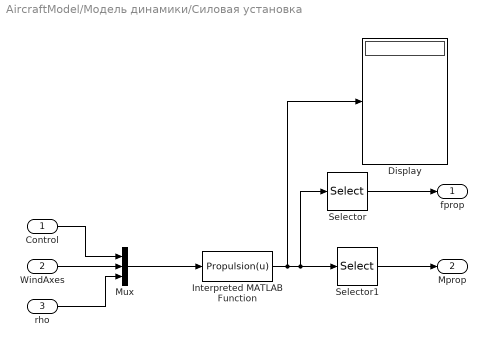
== system AircraftModel/Модель динамики/Силовая установка ==
  Control : Inport
  WindAxes : Inport  Port=2
  rho : Inport  Port=3
  Display : Display
  Interpreted MATLAB Function : MATLABFcn  MATLABFcn=Propulsion(u)  OutputDimensions=6
  Mux : Mux  Inputs=3
  Selector : Selector  InputPortWidth=6  IndexOptions=Index vector (dialog)  Indices=[1 2 3]  OutputSizes=1
  Selector1 : Selector  InputPortWidth=6  IndexOptions=Index vector (dialog)  Indices=[4 5 6]  OutputSizes=1
  fprop : Outport
  Mprop : Outport  Port=2
  wires:
  Control/1 -> Mux/1
  WindAxes/1 -> Mux/2
  Mux/1 -> Interpreted MATLAB Function/1
  Interpreted MATLAB Function/1 -> Selector1/1, Selector/1, Display/1
  rho/1 -> Mux/3
  Selector/1 -> fprop/1
  Selector1/1 -> Mprop/1

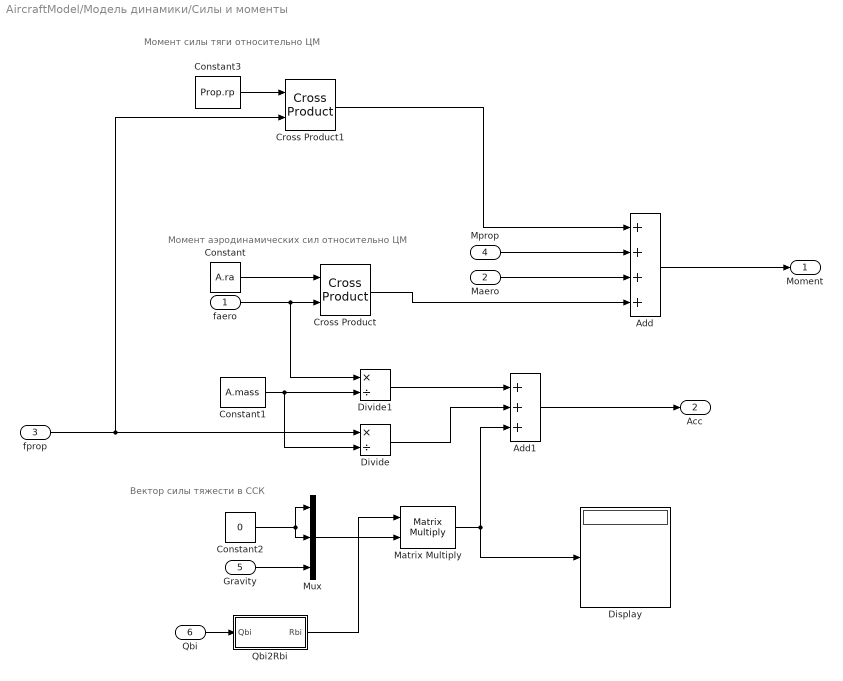
== system AircraftModel/Модель динамики/Силы и моменты ==
  note: Момент силы тяги относительно ЦМ
  note: Вектор силы тяжести в ССК
  note: Момент аэродинамических сил относительно ЦМ
  faero : Inport
  Maero : Inport  Port=2
  fprop : Inport  Port=3
  Mprop : Inport  Port=4
  Gravity : Inport  Port=5
  Qbi : Inport  Port=6
  Add : Sum  Inputs=++++
  Add1 : Sum  Inputs=+++
  Constant : Constant  Value=A.ra
  Constant1 : Constant  Value=A.mass
  Constant2 : Constant  Value=0
  Constant3 : Constant  Value=Prop.rp
  Cross Product : matrix_library/Cross Product
  Cross Product1 : matrix_library/Cross Product
  Display : Display
  Divide : Product  Inputs=*/
  Divide1 : Product  Inputs=*/
  Matrix Multiply : Product  Multiplication=Matrix(*)
  Mux : Mux  Inputs=3
  Qbi2Rbi : Subsystem
  Moment : Outport
  Acc : Outport  Port=2
  wires:
  faero/1 -> Cross Product/2, Divide1/1
  Maero/1 -> Add/3
  Gravity/1 -> Mux/3
  Mprop/1 -> Add/2
  fprop/1 -> Cross Product1/2, Divide/1
  Add/1 -> Moment/1
  Constant/1 -> Cross Product/1
  Cross Product/1 -> Add/4
  Add1/1 -> Acc/1
  Constant1/1 -> Divide/2, Divide1/2
  Divide1/1 -> Add1/1
  Divide/1 -> Add1/2
  Constant2/1 -> Mux/1, Mux/2
  Mux/1 -> Matrix Multiply/2
  Qbi2Rbi/1(Rbi) -> Matrix Multiply/1
  Matrix Multiply/1 -> Add1/3, Display/1
  Qbi/1 -> Qbi2Rbi/1(Qbi)
  Constant3/1 -> Cross Product1/1
  Cross Product1/1 -> Add/1

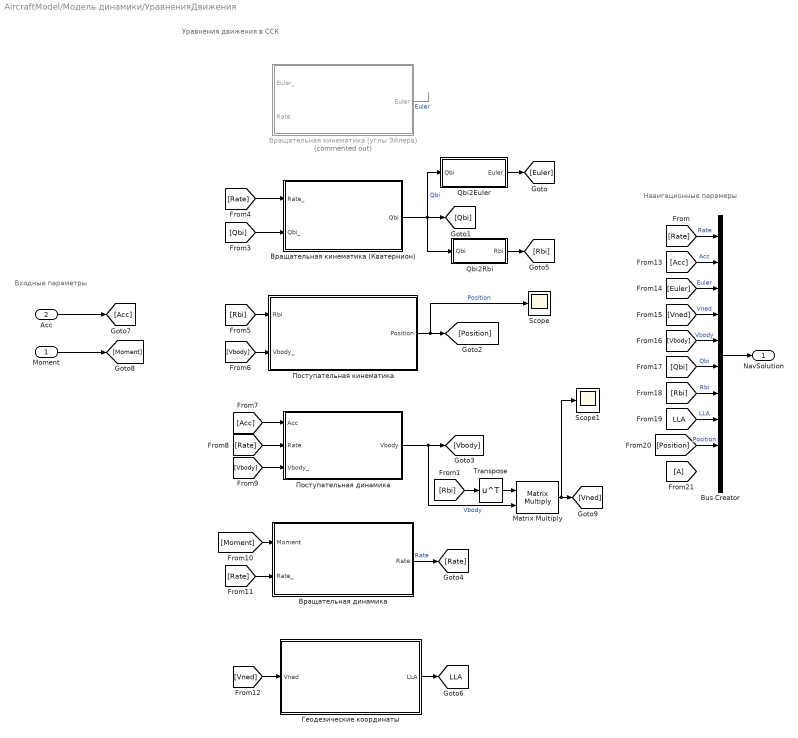
== system AircraftModel/Модель динамики/УравненияДвижения ==
  note: Уравнения движения в ССК
  note: Входные параметры
  note: Навигационные парамеры
  " Moment" : Inport
  " Acc" : Inport  Port=2
  Bus Creator : BusCreator  Inputs=10
  From21 : From
  Matrix Multiply : Product  Multiplication=Matrix(*)
  Qbi2Euler : Subsystem
  Qbi2Rbi : Subsystem
  Scope : Scope
      settings: ActiveDisplayYMinimum=-1  ActiveDisplayYMaximum=1  DataLoggingVariableName=ScopeData2
  Scope1 : Scope
      settings: ActiveDisplayYMinimum=-1  ActiveDisplayYMaximum=1  DataLoggingVariableName=ScopeData3
  Transpose : Math  Operator=transpose
  Вращательная динамика : Subsystem
  Вращательная кинематика (Кватернион) : Subsystem
  Вращательная кинематика (углы Эйлера) : Subsystem  Commented=on
  Геодезические координаты : Subsystem
  Поступательная динамика : Subsystem
  Поступательная кинематика : Subsystem
  NavSolution : Outport
  tag scope: LLA=global
  wires:
  Bus Creator/1 -> NavSolution/1
  Вращательная кинематика (углы Эйлера)/1(Euler) -> ?  "Euler"
  Вращательная кинематика (Кватернион)/1(Qbi) -> [Qbi], Qbi2Rbi/1(Qbi), Qbi2Euler/1(Qbi)  "Qbi"
  Поступательная кинематика/1(Position) -> Scope/1, [Position]  "Position"
  Поступательная динамика/1(Vbody) -> [Vbody], Matrix Multiply/2  "Vbody"
  Вращательная динамика/1(Rate) -> [Rate]  "Rate"
  Qbi2Euler/1(Euler) -> [Euler]
  Qbi2Rbi/1(Rbi) -> [Rbi]
  [Rbi] -> Transpose/1
  Transpose/1 -> Matrix Multiply/1
  Геодезические координаты/1(LLA) -> [LLA]
  " Acc"/1 -> [Acc]
  " Moment"/1 -> [Moment]
  Matrix Multiply/1 -> Scope1/1, [Vned]
  [Qbi] -> Вращательная кинематика (Кватернион)/2(Qbi_)
  [Rate] -> Вращательная кинематика (Кватернион)/1(Rate_)
  [Rbi] -> Поступательная кинематика/1(Rbi)
  [Vbody] -> Поступательная кинематика/2(Vbody_)
  [Acc] -> Поступательная динамика/1(Acc)
  [Rate] -> Поступательная динамика/2(Rate)
  [Vbody] -> Поступательная динамика/3(Vbody_)
  [Moment] -> Вращательная динамика/1(Moment)
  [Rate] -> Вращательная динамика/2(Rate_)
  [Vned] -> Геодезические координаты/1(Vned)
  [Vbody] -> Bus Creator/5  "Vbody"
  [Position] -> Bus Creator/9  "Position"
  [LLA] -> Bus Creator/8  "LLA"
  [Rbi] -> Bus Creator/7  "Rbi"
  [Qbi] -> Bus Creator/6  "Qbi"
  [Vned] -> Bus Creator/4  "Vned"
  [Euler] -> Bus Creator/3  "Euler"
  [Acc] -> Bus Creator/2  "Acc"
  [Rate] -> Bus Creator/1  "Rate"

== system AircraftModel/Модель динамики/Силы и моменты/Qbi2Rbi ==
  Qbi : Inport
  Interpreted MATLAB Function : MATLABFcn  MATLABFcn=Qbi2Rbi(u)  OutputSignalType=real  Output1D=off
  Rbi : Outport
  wires:
  Qbi/1 -> Interpreted MATLAB Function/1
  Interpreted MATLAB Function/1 -> Rbi/1

== system AircraftModel/Модель динамики/УравненияДвижения/Qbi2Euler ==
  Qbi : Inport
  Interpreted MATLAB Function : MATLABFcn  MATLABFcn=Qbi2Euler(u)  OutputDimensions=3
  Euler : Outport
  wires:
  Qbi/1 -> Interpreted MATLAB Function/1
  Interpreted MATLAB Function/1 -> Euler/1

== system AircraftModel/Модель динамики/УравненияДвижения/Qbi2Rbi ==
  Qbi : Inport
  Interpreted MATLAB Function : MATLABFcn  MATLABFcn=Qbi2Rbi(u)  Output1D=off
  Rbi : Outport
  wires:
  Qbi/1 -> Interpreted MATLAB Function/1
  Interpreted MATLAB Function/1 -> Rbi/1

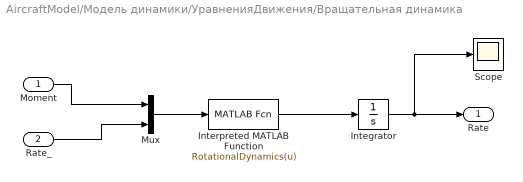
== system AircraftModel/Модель динамики/УравненияДвижения/Вращательная динамика ==
  Moment : Inport
  Rate_ : Inport  Port=2
  Integrator : Integrator  InitialCondition=InitRate
  Interpreted MATLAB Function : MATLABFcn  MATLABFcn=RotationalDynamics(u)
  Mux : Mux  Inputs=2
  Scope : Scope
      settings: ActiveDisplayYMinimum=-1.6077112404744893  ActiveDisplayYMaximum=2.1231850151588181
  Rate : Outport
  wires:
  Moment/1 -> Mux/1
  Interpreted MATLAB Function/1 -> Integrator/1
  Mux/1 -> Interpreted MATLAB Function/1
  Rate_/1 -> Mux/2
  Integrator/1 -> Scope/1, Rate/1

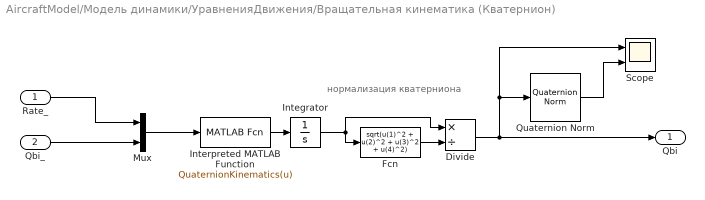
== system AircraftModel/Модель динамики/УравненияДвижения/Вращательная кинематика (Кватернион) ==
  note: нормализация кватерниона
  Rate_ : Inport
  Qbi_ : Inport  Port=2
  Divide : Product  Inputs=*/
  Fcn : Fcn  Expr=sqrt(u(1)^2 + u(2)^2 + u(3)^2 + u(4)^2)
  Integrator : Integrator  InitialCondition=Euler2Qbi(InitEuler)
  Interpreted MATLAB Function : MATLABFcn  MATLABFcn=QuaternionKinematics(u)
  Mux : Mux  Inputs=2
  Quaternion Norm : sharedutil/Quaternion Norm  aMode=aMode
      settings: LibrarySourceBlock=|
      | aerolibutil/Quaternion
      | Norm
  Scope : Scope  NumInputPorts=2
      settings: ActiveDisplayYMinimum=-1.2497875856171963  ActiveDisplayYMaximum=1.249976398401911
  Qbi : Outport
  wires:
  Rate_/1 -> Mux/1
  Integrator/1 -> Divide/1, Fcn/1
  Interpreted MATLAB Function/1 -> Integrator/1
  Mux/1 -> Interpreted MATLAB Function/1
  Qbi_/1 -> Mux/2
  Fcn/1 -> Divide/2
  Divide/1 -> Quaternion Norm/1, Scope/1, Qbi/1
  Quaternion Norm/1 -> Scope/2

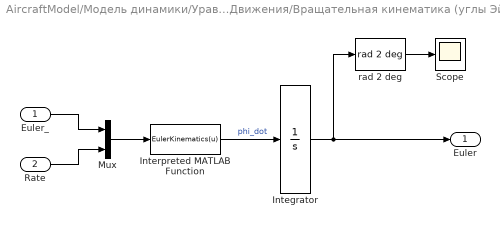
== system AircraftModel/Модель динамики/УравненияДвижения/Вращательная кинематика (углы Эйлера) ==
  " Euler_" : Inport
  Rate : Inport  Port=2
  Integrator : Integrator  InitialCondition=[0;0;0]
  Interpreted MATLAB Function : MATLABFcn  MATLABFcn=EulerKinematics(u)
  Mux : Mux  Inputs=2
  Scope : Scope
      settings: ActiveDisplayYMinimum=-73.780300166117428  ActiveDisplayYMaximum=225.35948699818604
  rad 2 deg : aerosimlib/Unit Conversion/Angular position/rad 2 deg
      settings: SourceProductName=AeroSim Blockset
  Euler : Outport
  wires:
  " Euler_"/1 -> Mux/1
  Rate/1 -> Mux/2
  Mux/1 -> Interpreted MATLAB Function/1
  Interpreted MATLAB Function/1 -> Integrator/1  "phi_dot"
  Integrator/1 -> Euler/1, rad 2 deg/1
  rad 2 deg/1 -> Scope/1

== system AircraftModel/Модель динамики/УравненияДвижения/Геодезические координаты ==
  Vned : Inport
  Integrator : Integrator  InitialCondition=InitLLA
  Interpreted MATLAB Function : MATLABFcn  MATLABFcn=Coordinates(u)
  Mux : Mux
  LLA : Outport
  wires:
  Vned/1 -> Mux/1
  [Rm] -> Mux/2
  [Rn] -> Mux/3
  Mux/1 -> Interpreted MATLAB Function/1
  Interpreted MATLAB Function/1 -> Integrator/1
  Integrator/1 -> Mux/4, LLA/1

== system AircraftModel/Модель динамики/УравненияДвижения/Поступательная динамика ==
  Acc : Inport
  Rate : Inport  Port=2
  Vbody_ : Inport  Port=3
  Add : Sum
  Cross Product : matrix_library/Cross Product
  Integrator : Integrator  InitialCondition=InitVbody
  Vbody : Outport
  wires:
  Acc/1 -> Add/2
  Rate/1 -> Cross Product/2
  Vbody_/1 -> Cross Product/1
  Cross Product/1 -> Add/1
  Add/1 -> Integrator/1
  Integrator/1 -> Vbody/1

== system AircraftModel/Модель динамики/УравненияДвижения/Поступательная кинематика ==
  Rbi : Inport
  Vbody_ : Inport  Port=2
  Integrator : Integrator  InitialCondition=[0;0;0]
  Matrix Multiply : Product  Multiplication=Matrix(*)
  Transpose : Math  Operator=transpose
  Position : Outport
  wires:
  Rbi/1 -> Transpose/1
  Vbody_/1 -> Matrix Multiply/2
  Matrix Multiply/1 -> Integrator/1
  Transpose/1 -> Matrix Multiply/1
  Integrator/1 -> Position/1
